simulink model "UDB4_TestBoard"  (Simulink 7.8)
settings: Solver=FixedStepDiscrete  SolverMode=SingleTasking  StartTime=0.0  StopTime=inf  FixedStep=0.001  RelTol=1e-3
libraries: dsPICdrivers x11, simulink x6
settings Model: Creator=Lior  LastModifiedBy=M91449  BufferReuse=off
settings OptimizationCC: BlockReduction=off  InlineParams=on  BufferReuse=off  OptimizeModelRefInitCode=on  LifeSpan=1
settings DebuggingCC: FcnCallInpInsideContextMsg=Use local settings
settings HardwareCC: ProdBitPerInt=16  ProdBitPerPointer=16  ProdEndianess=LittleEndian  ProdWordSize=16  ProdHWDeviceType=16-bit Generic
settings RTWCC: SystemTargetFile=dspic.tlc  MakeCommand=make_CreateMPLAB  TemplateMakefile=dspic_pic30_gcc.tmf  PostCodeGenCommand=dsPIC_Compile()  Description=Embedded Target for Microchip dsPIC (real-time)  ProcessScript=dspic_make_rtw_hook
settings CodeAppCC: IgnoreCustomStorageClasses=off
settings STFCustomTargetCC: IncludeMdlTerminateFcn=off  GeneratePreprocessorConditionals=Use local settings  CombineOutputUpdateFcns=on  SuppressErrorStatus=on  ERTCustomFileBanners=on  SupportContinuousTime=off  SupportNonInlinedSFcns=off  SystemTargetFile=dspic.tlc
settings ERTTargetCC: MultiwordLength=2048  ParMdlRefBuildCompliant=off  CompOptLevelCompliant=off  ConcurrentExecutionCompliant=off  IncludeMdlTerminateFcn=off  SuppressErrorStatus=on  ERTFirstTimeCompliant=off  ModelStepFunctionPrototypeControlCompliant=off  CPPClassGenCompliant=off  ExtModeMexFile=noextcomm  InlinedParameterPlacement=NonHierarchical  ERTSrcFileBannerTemplate=dsPIC_code_template.cgt  ERTHdrFileBannerTemplate=dsPIC_code_template.cgt  ERTDataSrcFileTemplate=dsPIC_code_template.cgt  ERTDataHdrFileTemplate=dsPIC_code_template.cgt  ERTCustomFileTemplate=dsPIC_main.tlc  ConvertIfToSwitch=off  SuppressUnreachableDefaultCases=off
settings CustomProperty: DataType=string  Value=C:\PROGRA~1\MATLAB\R2011B~1\bin\win64\gmake

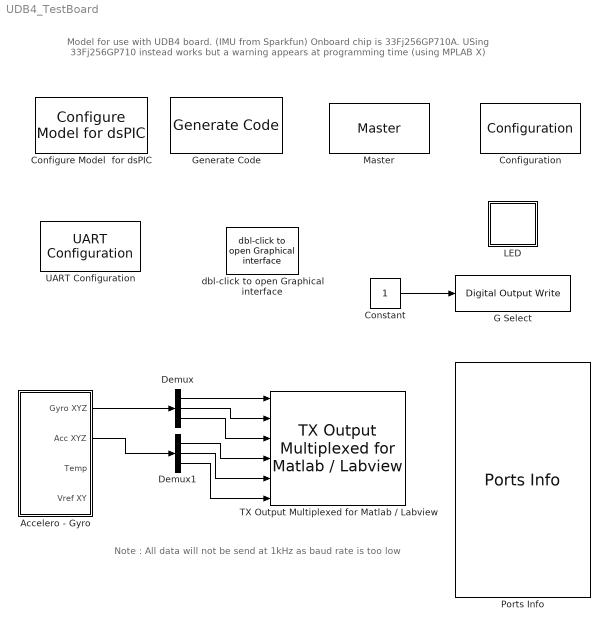
== system UDB4_TestBoard ==
  note: Model for use with UDB4 board. (IMU from Sparkfun)
      | Onboard chip is 33Fj256GP710A.
      | USing 33Fj256GP710 instead works but a warning appears at programming time (using MPLAB X)
  note: Note : All data will not be send at 1kHz as baud rate is too low
  Accelero - Gyro : Subsystem
  Configuration : dsPICdrivers/Configuration  double64=off
  Configure Model  for dsPIC : dsPICdrivers/Simulink Configuration/Configure Model  for dsPIC
  Constant : Constant  OutDataTypeStr=Inherit: Inherit via back propagation
  Demux : Demux  Outputs=3
  Demux1 : Demux  Outputs=3
  G Select : dsPICdrivers/Digital I//O/Digital Output Write  Tag=dsPIC_Digital_Output  Priority=5  PORT=A  Pin=6  Simultaneous=on  OrderingInOutPopup=None
  Generate Code : dsPICdrivers/Simulink Configuration/Generate Code
  LED : Subsystem
  Master : dsPICdrivers/Master  Tag=dsPIC_MASTER  Priority=1  TimeStepType=Timer1  picType=33fJ256GP710  fcy=7375000  Quartz_33f=8e6  PLLActive_33f=on  fcyDesired_33f=7.37e6  tmr1="[1  7374  0]"  tmr1Info="Time Step : 0.001  ;   Error : 0%  PR1=7374"  tmr2345="[0  0  0  0  0  0  0  0]"  tmr2345cfg=[-1 -1 -1 -1 -1 -1 -1 -1]  IOautoConf=on  typePort="[ 0   0   0   0   0   0  10   0   0   0   0   0   0   0   0   0   8   8   0   8   8   8   8   8   0   8   8   8   8   0   0   0   0   0   0   0   0   0   0   0   0   0   0   0   0   0   0   0   0   0   0   0   0   0   0   0   0   0   0   0   0   0   0   0   0  10  10  10  10   0   0   0   0   0   0   0   0   0   0   0   0   0   0   0   4   5   0   0   0   0   0   0   0   0   0   0   0   0   0   0   0   0   0   0   0   0   0   0   0   0   0   0 ]"  TRIS="[ 65471  65535  65535  65535  65505  65535  65535 ]"  ADPCFG=507510784  MasterBusyPort=None  MasterOverloadPort=None  FOSC=Quartz (XT - HS)  ClockSwitchMonitor=Clock switching enabled only  TempProtection_33f=TEMP_ON  FPBOR=<empty>  PWRT=disable  MCLR=<empty>  ICD=ICS_PGD1  JTAGEN=JTAGEN_OFF  PowerSave=off  OverrideFcy=off  NewFcy=1e6  PR2345="[65535  65535  65535  65535  65535  65535  65535  65535]"
  Ports Info : dsPICdrivers/Ports Info  Tag=dsPIC_PortInfo
  TX Output Multiplexed for Matlab / Labview : dsPICdrivers/Serial PORT/TX Output Multiplexed for Matlab // Labview  Tag=dsPIC_TX_Multiplexed  Priority=5  UART=2  CleverSpreadingChk=on  CleverSpreading=1  CHANNEL=[0:5]  CHANNELBLOCKED=[]  CHANNELBLOCKED_BITEWISE=0  Status=OK
  UART Configuration : dsPICdrivers/Serial PORT/UART Configuration  Tag=dsPIC_config_UART  Priority=2  UART=2  proposed_BAUD=Custom  BAUD=115200  ALT_TX_RX=on  InterruptTxWhen=When Transmit Buffer is empty  TXInterruptPri=1  TxBufferSize=32  TXEN=on  InterruptRxWhen=When Receive Buffer is full (contain 4 characters)  RXInterruptPri=2  RxBufferSize=32  DoNotImplementRxInterrupt=off  DoNotImplementTxInterrupt=off  UxBRG=3  Info="UxBRG = 3   ||  Real Baud : 115234   ||  % error : 0.029839  ||  max 11.5234 Bytes / Step"  RealBaud=0  ERROR=0.029839  BYTES_STEP=11.5234
  dbl-click to open Graphical interface : dsPICdrivers/Serial PORT/dbl-click to open Graphical interface  Nothing=0
  wires:
  Constant/1 -> G Select/1
  Accelero - Gyro/1(Gyro XYZ) -> Demux/1
  Accelero - Gyro/2(Acc XYZ) -> Demux1/1
  Demux/1 -> TX Output Multiplexed for Matlab / Labview/1
  Demux/2 -> TX Output Multiplexed for Matlab / Labview/2
  Demux/3 -> TX Output Multiplexed for Matlab / Labview/3
  Demux1/1 -> TX Output Multiplexed for Matlab / Labview/4
  Demux1/2 -> TX Output Multiplexed for Matlab / Labview/5
  Demux1/3 -> TX Output Multiplexed for Matlab / Labview/6

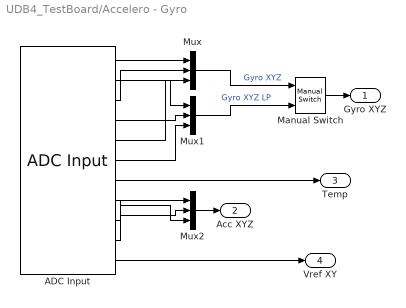
== system UDB4_TestBoard/Accelero - Gyro ==
  ADC Input : dsPICdrivers/Peripheral I//O/ADC Input  Tag=dsPIC_ADC  Priority=5  ADC_TYPE=12 bits  ADC_MODE=Continuous sampling & get last channel value  NbrSampleStep=1  VoltRefpopup="AVdd  -  AVss"  OutFormatBitspopup=0000 dddd dddd dddd : Integer  InterruptPriority=6  ANCHANNELS=[9 10 11 12 0 1 3 4 5 6 7]  MaxName=ANmax = 4095  Rin=1e2  ADCS=9  SAMC=1  Temperature=25  DMAChannel=0  SampleTime=.001  Status="OK  |  Tsmp=6.780e-007 |  T/Channel=1.017e-005 |  Tall=1.119e-004"  SSRC=auto convert
  Manual Switch : simulink/Signal Routing/Manual Switch  sw=1  action=0  varsize=off
  Mux : Mux  Inputs=3
  Mux1 : Mux  Inputs=3
  Mux2 : Mux  Inputs=3
  Gyro XYZ : Outport
  Acc XYZ : Outport  Port=2
  Temp : Outport  Port=3
  Vref XY : Outport  Port=4
  wires:
  ADC Input/1 -> Mux/1
  ADC Input/3 -> Mux/2
  ADC Input/5 -> Mux/3
  ADC Input/2 -> Mux1/1
  ADC Input/4 -> Mux1/2
  ADC Input/6 -> Mux1/3
  ADC Input/10 -> Mux2/1
  ADC Input/9 -> Mux2/2
  ADC Input/8 -> Mux2/3
  Mux/1 -> Manual Switch/1  "Gyro XYZ"
  Mux1/1 -> Manual Switch/2  "Gyro XYZ LP"
  Manual Switch/1 -> Gyro XYZ/1
  ADC Input/7 -> Temp/1
  Mux2/1 -> Acc XYZ/1
  ADC Input/11 -> Vref XY/1

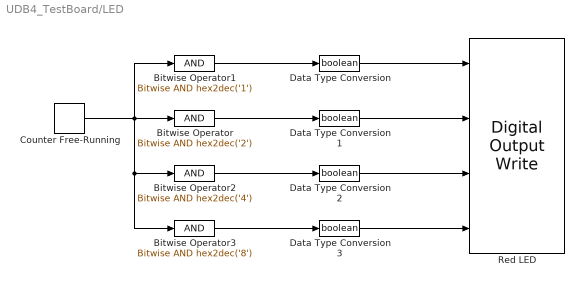
== system UDB4_TestBoard/LED ==
  Bitwise Operator : simulink/Logic and Bit Operations/Bitwise Operator  logicop=AND  UseBitMask=on  BitMask=hex2dec('2')  BitMaskRealWorld=Stored Integer
  Bitwise Operator1 : simulink/Logic and Bit Operations/Bitwise Operator  logicop=AND  UseBitMask=on  BitMask=hex2dec('1')  BitMaskRealWorld=Stored Integer
  Bitwise Operator2 : simulink/Logic and Bit Operations/Bitwise Operator  logicop=AND  UseBitMask=on  BitMask=hex2dec('4')  BitMaskRealWorld=Stored Integer
  Bitwise Operator3 : simulink/Logic and Bit Operations/Bitwise Operator  logicop=AND  UseBitMask=on  BitMask=hex2dec('8')  BitMaskRealWorld=Stored Integer
  Counter Free-Running : simulink/Sources/Counter Free-Running  NumBits=4  tsamp=.1
  Data Type Conversion{,1..3} (4 alike) : DataTypeConversion  OutDataTypeStr=boolean
  Red LED : dsPICdrivers/Digital I//O/Digital Output Write  Tag=dsPIC_Digital_Output  Priority=5  PORT=E  Pin=[1 2 3 4]  Simultaneous=on  OrderingInOutPopup=None
  wires:
  Data Type Conversion/1 -> Red LED/1
  Data Type Conversion1/1 -> Red LED/2
  Data Type Conversion2/1 -> Red LED/3
  Data Type Conversion3/1 -> Red LED/4
  Bitwise Operator1/1 -> Data Type Conversion/1
  Bitwise Operator/1 -> Data Type Conversion1/1
  Bitwise Operator2/1 -> Data Type Conversion2/1
  Bitwise Operator3/1 -> Data Type Conversion3/1
  Counter Free-Running/1 -> Bitwise Operator/1, Bitwise Operator1/1, Bitwise Operator2/1, Bitwise Operator3/1
